simulink model "turbo_controller"  (R2025a)
settings: Solver=FixedStepAuto  StartTime=0.0  StopTime=inf  FixedStep=0.001  RelTol=1e-3
PostLoadFcn:
  | % 自动定位同目录CubeMX文件；不需要外部初始化脚本。
  | codertarget.data.setParameterValue('turbo_controller','STM32CubeMX.ProjectFile',fullfile(fileparts(get_param('turbo_controller','FileName')),'turbo_f407.ioc'));
InitFcn:
  | % 中文说明：按原控制器字段与类型创建三组接口总线；控制参数已内嵌。
  | tc_names=["EValve_Cycle" "EValve_Open" "Eblast_Cycle" "Eblast_Open" "Motor_Cycle" "Motor_Open" "EValve_Enable" "Eblast_Enable" "Motor_Enable" "SWO_Firework" "SWO_BleedAir" "EngineState" "Flag_ECUReset_Clear" "Flag_ECUReset_Save" "Flag_Reset_Enable" "Accelerator" "Nc_dem" "Nc"]; tc_types=["uint16" "uint16" "uint16" "uint16" "uint16" "uint16" "uint8" "uint8" "uint8" "uint8" "uint8" "uint8" "uint8" "uint8" "uint8" "single" "single" "single"];
  | for tc_k=1:numel(tc_names)
  |  tc_e(tc_k)=Simulink.BusElement; tc_e(tc_k).Name=char(tc_names(tc_k)); tc_e(tc_k).DataType=char(tc_types(tc_k));
  | end
  | EngineControl_Out=Simulink.Bus; EngineControl_Out.DataScope='Exported'; EngineControl_Out.Elements=tc_e;
  | clear tc_e tc_names tc_types tc_k
  | tc_names=["savedata1" "savedata2" "savedata3" "savedata4" "savedata5" "savedata6" "savedata7" "savedata8" "savedata9" "savedata10" "savedata11" "savedata12" "savedata13" "savedata14" "savedata15" "savedata16" "savedata17" "savedata18" "savedata19" "savedata20" "savedata21" "savedata22" "savedata23" "savedata24" "savedata25"]; tc_types=["single" "single" "single" "single" "single" "single" "single" "single" "single" "single" "single" "single" "single" "single" "single" "single" "single" "single" "single" "single" "single" "single" "single" "single" "single"];
  | for tc_k=1:numel(tc_names)
  |  tc_e(tc_k)=Simulink.BusElement; tc_e(tc_k).Name=char(tc_names(tc_k)); tc_e(tc_k).DataType=char(tc_types(tc_k));
  | end
  | SaveData_Out=Simulink.Bus; SaveData_Out.DataScope='Exported'; SaveData_Out.Elements=tc_e;
  | clear tc_e tc_names tc_types tc_k
  | tc_names=["senddata1" "senddata2" "senddata3" "senddata4" "senddata5" "senddata6" "senddata7" "senddata8" "senddata9" "senddata10" "senddata11" "senddata12" "senddata13" "senddata14" "senddata15" "senddata16" "senddata17" "senddata18" "senddata19" "senddata20" "senddata21" "senddata22" "senddata23" "senddata24" "senddata25" "senddata26" "senddata27" "senddata28" "senddata29"]; tc_types=["uint8" "uint8" "uint8" "uint8" "uint8" "uint8" "uint8" "uint8" "uint8" "uint8" "uint8" "uint8" "uint8" "uint8" "uint8" "uint8" "uint8" "uint8" "uint8" "uint8" "uint8" "uint8" "uint8" "uint8" "uint8" "uint8" "uint8" "uint8" "uint8"];
  | for tc_k=1:numel(tc_names)
  |  tc_e(tc_k)=Simulink.BusElement; tc_e(tc_k).Name=char(tc_names(tc_k)); tc_e(tc_k).DataType=char(tc_types(tc_k));
  | end
  | SendData_Out=Simulink.Bus; SendData_Out.DataScope='Exported'; SendData_Out.Elements=tc_e;
  | clear tc_e tc_names tc_types tc_k
  | 
  | % 以下为接口中文说明；只设置描述，不改变数值或数据类型。
  | EngineControl_Out.Description='执行控制输出（阀、电机、点火、状态及复位请求）';
  | tc_cn=["EValve_Cycle（主油阀周期计数（每计数2毫秒））" "EValve_Open（主油阀开通计数（每计数2毫秒））" "Eblast_Cycle（副油阀周期计数（每计数2毫秒））" "Eblast_Open（副油阀开通计数（每计数2毫秒））" "Motor_Cycle（起动电机周期计数）" "Motor_Open（起动电机开通计数）" "EValve_Enable（主油阀驱动使能）" "Eblast_Enable（副油阀驱动使能）" "Motor_Enable（起动电机使能）" "SWO_Firework（点火器使能（1开））" "SWO_BleedAir（引气阀使能（1开））" "EngineState（发动机状态）" "Flag_ECUReset_Clear（清除复位恢复状态请求）" "Flag_ECUReset_Save（保存复位恢复数据请求）" "Flag_Reset_Enable（处理器软件复位请求）" "Accelerator（油门／油泵给定控制量）" "Nc_dem（控制目标转速）" "Nc（发动机反馈转速（转每分））"];
  | tc_elements=EngineControl_Out.Elements;
  | for tc_k=1:numel(tc_cn)
  |  tc_elements(tc_k).Description=char(tc_cn(tc_k));
  | end
  | EngineControl_Out.Elements=tc_elements;
  | clear tc_cn tc_elements tc_k
  | SaveData_Out.Description='25项运行记录；字段含义按当前模型数据来源解释';
  | tc_cn=["savedata1（指令回显记录）" "savedata2（入口总温记录（℃））" "savedata3（电源电压记录）" "savedata4（排气温度记录（℃））" "savedata5（标定燃油压力记录）" "savedata6（副油阀占空比记录（％））" "savedata7（主油阀占空比记录（％））" "savedata8（温度修正转速记录）" "savedata9（开关输出及反馈位域）" "savedata10（物理转速记录）" "savedata11（油泵目标给定原始值）" "savedata12（起动电机占空比记录（％））" "savedata13（发动机状态码记录）" "savedata14（故障告警位域记录）" "savedata15（模型记录帧序号）" "savedata16（处理器温度记录（℃））" "savedata17（装订转速记录（沿用旧电源字段名））" "savedata18（导航高度记录）" "savedata19（飞行空速记录）" "savedata20（主阀旧记录位（恒零保留））" "savedata21（第21项保留记录（恒零））" "savedata22（保留记录项22）" "savedata23（保留记录项23）" "savedata24（保留记录项24）" "savedata25（保留记录项25）"];
  | tc_elements=SaveData_Out.Elements;
  | for tc_k=1:numel(tc_cn)
  |  tc_elements(tc_k).Description=char(tc_cn(tc_k));
  | end
  | SaveData_Out.Elements=tc_elements;
  | clear tc_cn tc_elements tc_k
  | SendData_Out.Description='29字段回传及外设命令接口；板端上位机帧只取第3至27字段';
  | tc_cn=["senddata1（回传发送允许标志（不直接上线路））" "senddata2（回传载荷长度25字节）" "senddata3（回传指令回显字节）" "senddata4（总温编码字节（℃＋80））" "senddata5（电源电压编码字节）" "senddata6（排温编码高字节）" "senddata7（排温编码低字节）" "senddata8（燃油压力编码高字节）" "senddata9（燃油压力编码低字节）" "senddata10（副油阀占空比字节（％））" "senddata11（主油阀占空比字节（％））" "senddata12（修正转速编码高字节）" "senddata13（修正转速编码低字节）" "senddata14（驱动及反馈状态位域）" "senddata15（物理转速编码高字节）" "senddata16（物理转速编码低字节）" "senddata17（油泵目标给定高字节（串口二使用））" "senddata18（油泵目标给定低字节（串口二使用））" "senddata19（起动电机占空比命令（串口一使用））" "senddata20（发动机状态码字节）" "senddata21（故障告警位域字节）" "senddata22（帧序号占位（板端另行填写））" "senddata23（处理器温度编码（℃＋50））" "senddata24（控制目标转速编码高字节）" "senddata25（控制目标转速编码低字节）" "senddata26（占位字节（板端改填实测泵速高字节））" "senddata27（占位字节（板端改填实测泵速低字节））" "senddata28（装订转速高字节（本板未发送））" "senddata29（装订转速低字节（本板未发送））"];
  | tc_elements=SendData_Out.Elements;
  | for tc_k=1:numel(tc_cn)
  |  tc_elements(tc_k).Description=char(tc_cn(tc_k));
  | end
  | SendData_Out.Elements=tc_elements;
  | clear tc_cn tc_elements tc_k
  | 
  | 
  | % FRAM模块化事务：接口类型和上电初始状态，随模型保存，无外部初始化文件。
  | clear FM_elements
  | FM_elements(1)=Simulink.BusElement;FM_elements(1).Name='phase';FM_elements(1).DataType='uint8';FM_elements(1).Dimensions=[1 1];FM_elements(1).Description='phase（当前事务阶段）';
  | FM_elements(2)=Simulink.BusElement;FM_elements(2).Name='a';FM_elements(2).DataType='uint8';FM_elements(2).Dimensions=[64 1];FM_elements(2).Description='a（启动时缓存的首区64字节）';
  | FM_elements(3)=Simulink.BusElement;FM_elements(3).Name='active';FM_elements(3).DataType='uint16';FM_elements(3).Dimensions=[1 1];FM_elements(3).Description='active（当前有效记录区地址）';
  | FM_elements(4)=Simulink.BusElement;FM_elements(4).Name='generation';FM_elements(4).DataType='uint32';FM_elements(4).Dimensions=[1 1];FM_elements(4).Description='generation（当前有效记录代号）';
  | FM_elements(5)=Simulink.BusElement;FM_elements(5).Name='record';FM_elements(5).DataType='uint8';FM_elements(5).Dimensions=[64 1];FM_elements(5).Description='record（本次冻结的待写记录）';
  | FM_elements(6)=Simulink.BusElement;FM_elements(6).Name='addr';FM_elements(6).DataType='uint16';FM_elements(6).Dimensions=[1 1];FM_elements(6).Description='addr（本次备用写入地址）';
  | FM_elements(7)=Simulink.BusElement;FM_elements(7).Name='lastSave';FM_elements(7).DataType='single';FM_elements(7).Dimensions=[1 1];FM_elements(7).Description='lastSave（上次开始保存的秒数）';
  | FM_elements(8)=Simulink.BusElement;FM_elements(8).Name='lastState';FM_elements(8).DataType='uint8';FM_elements(8).Dimensions=[1 1];FM_elements(8).Description='lastState（上次保存时的发动机状态）';
  | FM_elements(9)=Simulink.BusElement;FM_elements(9).Name='boot';FM_elements(9).DataType='boolean';FM_elements(9).Dimensions=[1 1];FM_elements(9).Description='boot（启动记录是否允许恢复）';
  | FM_elements(10)=Simulink.BusElement;FM_elements(10).Name='consumed';FM_elements(10).DataType='boolean';FM_elements(10).Dimensions=[1 1];FM_elements(10).Description='consumed（本次启动恢复通知是否已发送）';
  | FM_elements(11)=Simulink.BusElement;FM_elements(11).Name='payload';FM_elements(11).DataType='uint8';FM_elements(11).Dimensions=[20 1];FM_elements(11).Description='payload（当前20字节恢复内容）';
  | ... (+35 lines)
model workspace (MAT data in the model file):
  CRC16_Table_Reference = [0 4129 8258 12387 16516 20645 24774 28903 33032 37161 41290 45419 ... (256 elements, 256x1)]
  PE_Kaer = [0.15402 0.15402 0.12264 0.10076 0.09481 0.07601 0.07111 0.0569 0.05198 0.04926 0.05308 0.04325 ... (13 elements, 1x13)]
  PE_Nr = [21.2982 61.4260372 67.7475458 72.7394382 76.845934 80.6988798 83.8449282 86.6491912 88.9382406 89.178606 91.1938214 93.4068058 ... (13 elements, 1x13)]
  PE_Pump_Translate = 33.5999984741
  PE_RotaSpeed_Translate = 860
  PE_Taer = [0.4939154 0.4939154 0.40780982 0.34066978 0.31622756 0.30405716 0.34300244 0.26785022 0.37393554 0.23914836 0.44563948 0.31044662 ... (13 elements, 1x13)]
  PF_ACCFULLRANGE = 3360
  PF_Flag_ECUReset = 0
  PF_Flag_rx_suc = 1
  PF_Gear_Info = [40000; 45000; 50000; 55000; 57000; 59000; 60000; 61000; 61000; 61000; 61000; 61000]
  PF_K_TiaoJie = 1
  PF_Kpu = 10
  PF_MySet_Rxdata = [0 0 0 0 0 0 0 0 0 0 0 0 ... (50 elements, 50x1)]
  PF_MyUsart1_Rxdata = [0 0 0 0 0 0 0 0 0 0 0 0 ... (50 elements, 50x1)]
  PF_MyUsart2_Rxdata = [0 0 0 0 0 0 0 0 0 0 0 0 ... (50 elements, 50x1)]
  PF_Reset_Information = [0 0 0 0 0 0 0 0 0 0 0 0 ... (20 elements, 20x1)]
  PF_Sensor_X1_T4 = [0 4095]
  PF_Sensor_X2_T4 = [0 1.66666698456]
  PF_Sensor_X3_T4 = [0 504 999 1497 2010 2529 3051 3568 4076 4571 4959]
  PF_Sensor_X_P2 = [0.5 3]
  PF_Sensor_X_Poil = [0.5 3]
  PF_Sensor_X_T1t = [-50 300]
  PF_Sensor_X_Vpower = [0 3]
  PF_Sensor_X_Vpump = [0 3]
  PF_Sensor_Y1_T4 = [0 3]
  PF_Sensor_Y2_T4 = [0 5000]
  PF_Sensor_Y3_T4 = [0 100 200 300 400 500 600 700 800 900 980]
  PF_Sensor_Y_P2 = [0 1000]
  PF_Sensor_Y_Poil = [0 1000]
  PF_Sensor_Y_T1t = [-50 300]
  PF_Sensor_Y_Vpower = [0 33]
  PF_Sensor_Y_Vpump = [0 33]
  PG_CtrlMode_CloseLoop : mpt.Parameter (value not decoded)
  PG_CtrlMode_ManualAcc : mpt.Parameter (value not decoded)
  PG_CtrlMode_Origin : mpt.Parameter (value not decoded)
  PG_CtrlMode_Start : mpt.Parameter (value not decoded)
  PG_CtrlMode_Stop : mpt.Parameter (value not decoded)
  PG_ES_Clp : mpt.Parameter (value not decoded)
  PG_ES_EngStart : mpt.Parameter (value not decoded)
  PG_ES_Manual : mpt.Parameter (value not decoded)
  PG_ES_Origin : mpt.Parameter (value not decoded)
  PG_ES_Stop : mpt.Parameter (value not decoded)
  PG_Instr_BleedAirSet : mpt.Parameter (value not decoded)
  PG_Instr_CloseLoop : mpt.Parameter (value not decoded)
  PG_Instr_ECUReSet : mpt.Parameter (value not decoded)
  PG_Instr_EValveSet : mpt.Parameter (value not decoded)
  PG_Instr_EblastSet : mpt.Parameter (value not decoded)
  PG_Instr_Erase : mpt.Parameter (value not decoded)
  PG_Instr_FireWorkSet : mpt.Parameter (value not decoded)
  PG_Instr_ManualPlus : mpt.Parameter (value not decoded)
  PG_Instr_ManualrReduce : mpt.Parameter (value not decoded)
  PG_Instr_MotorSet : mpt.Parameter (value not decoded)
  PG_Instr_OilSet : mpt.Parameter (value not decoded)
  PG_Instr_SelfCheck : mpt.Parameter (value not decoded)
  PG_Instr_Start : mpt.Parameter (value not decoded)
  PG_Instr_Stop : mpt.Parameter (value not decoded)
  PG_Instr_StopZero : Simulink.Parameter (value not decoded)
  PG_Location_Air : Simulink.Parameter (value not decoded)
  PG_Location_Gnd : Simulink.Parameter (value not decoded)
  PG_ServoCtrlMode_CloseLoop : Simulink.Parameter (value not decoded)
  PG_ServoCtrlMode_CloseLoopMax : Simulink.Parameter (value not decoded)
  PG_ServoCtrlMode_CloseLoopMin : Simulink.Parameter (value not decoded)
  PG_ServoCtrlMode_ManualAcc : Simulink.Parameter (value not decoded)
  PG_ServoCtrlMode_ManualAccMax : Simulink.Parameter (value not decoded)
  PG_ServoCtrlMode_ManualAccMin : Simulink.Parameter (value not decoded)
  PG_SpeedDot_Permit : Simulink.Parameter (value not decoded)
  PL_EngineModel_Actuator = [0 10 100]
  PL_EngineModel_EngineStar_Press_P2 = [1013 1098.4 1099.144828 1099.931034 1103.613793 1162.662069 1143.793103 1131.006897 1123.186207 1117.6 1114 1111.806897 ... (127 elements, 1x127)]
  PL_EngineModel_EngineStar_RotaSpeed = [200 2000 9584 9660 10220 10240 10260 10288 10308 10368 10380 10408 ... (127 elements, 1x127)]
  PL_EngineModel_EngineStar_Temp_Exhaust = [128 129 129.1 130 131 131.1 132 133 134 134.1 135 135.1 ... (127 elements, 1x127)]
  PL_EngineModel_EngineStar_Time = [0.05 0.1 0.15 0.2 0.25 0.3 0.35 0.4 0.45 0.5 0.55 0.6 ... (127 elements, 1x127)]
  PL_EngineModel_IdleAbove_Nr = [0 21.2982 61.4260372 67.7475458 72.7394382 76.845934 80.6988798 83.8449282 86.6491912 88.9382406 89.178606 91.1938214 ... (14 elements, 1x14)]
  PL_EngineModel_IdleAbove_P2r = [0.986923266716 1.57907722675 1.81593881076 1.99358499877 2.23044658278 2.43770046879 2.65482358747 2.84233900814 3.03972366149 3.18776215149 3.25684678016 3.3950160375 ... (14 elements, 1x14)]
  PL_EngineModel_IdleAbove_Tempr = [0.0536001429337 1.07200285867 1.63301768805 1.63659103091 1.66875111667 1.72592460247 1.77595140254 1.86171163123 1.95461854565 2.03323208862 2.03323208862 2.13685903162 ... (14 elements, 1x14)]
  PL_EngineModel_IdleAbove_Ter = [0.42434128 0.42434128 0.42434128 0.30669408 0.23570008 0.22150128 0.1997974 0.23803274 0.16115638 0.24279948 0.13600422 0.31308354 ... (14 elements, 1x14)]
  PL_EngineModel_IdleAbove_Wfr = [0 10.142 23.8337 27.8905 31.9473 36.0041 40.0609 44.1177 48.1745 52.2313 52.7384 56.7952 ... (14 elements, 1x14)]
  PL_EngineModel_Press_P2 = [400 400 400 400 400 400 400 400 400 400]
  PL_EngineModel_Rotaspeed = [0 20000 96400]
  PL_EngineModel_Temp_Exhaust = [500 500 500 500 500 500 500 500 500 500]
  PL_Kaer = [0.1 0.1 0.1 0.1 0.1 0.1]
  PL_Nr = [50 60 70 80 90 100]
  PL_Taer = [0.1 0.1 0.1 0.1 0.1 0.1]
  Sig : Simulink.Signal (value not decoded)
  Ts_ms : Simulink.Parameter (value not decoded)
  false : Simulink.Parameter (value not decoded)
  true : Simulink.Parameter (value not decoded)
symbols that are objects in the model workspace (value not decoded): PG_CtrlMode_CloseLoop, PG_CtrlMode_ManualAcc, PG_CtrlMode_Origin, PG_CtrlMode_Start, PG_CtrlMode_Stop, PG_ES_Clp, PG_ES_EngStart, PG_ES_Manual, PG_ES_Origin, PG_ES_Stop, PG_Instr_BleedAirSet, PG_Instr_CloseLoop, PG_Instr_EblastSet, PG_Instr_ECUReSet, PG_Instr_Erase, PG_Instr_EValveSet, PG_Instr_FireWorkSet, PG_Instr_ManualPlus, PG_Instr_ManualrReduce, PG_Instr_MotorSet, PG_Instr_OilSet, PG_Instr_SelfCheck, PG_Instr_Start, PG_Instr_Stop, PG_Instr_StopZero, PG_ServoCtrlMode_CloseLoop, PG_ServoCtrlMode_CloseLoopMax, PG_ServoCtrlMode_CloseLoopMin, PG_ServoCtrlMode_ManualAcc, PG_ServoCtrlMode_ManualAccMax, PG_ServoCtrlMode_ManualAccMin, Ts_ms
libraries: simulink x97, stm32blockslib x10, stm32f4xxblockslib x8
(part 14 of 26)

== system turbo_controller/CLM/Manual/ManualAcc_Min_Control ==
  note: 形成手动油泵给定，并限制直接设定的范围
      |
      | 接收有效的手动直接设定命令时，把Data6限制在0～70，再乘以100，形成泵控制编码。例：Data6=35
      | 得到3500，Data6=90会先限制为70，输出7000。这是设备控制编码，不是油压或燃油流量。
      |
      | 没有直接设定命令时，使用“手动加减”分支产生的保持值。选择器决定采用新设定还是保持路径，范
      | 围模块防止结果超出允许值。对外同时给出手动控制上下界0和15000，供后续统一输出处理。最终泵命
      | 令还会经过使能、限幅和字节打包，才发送到泵。
  S_Flag_rs_suc : Inport
      settings: AttributesFormatString=S_Flag_rs_suc（标志接收状态成功或有效）
  S_Instr : Inport  Port=2
      settings: AttributesFormatString=S_Instr（指令）
  S_ServoOut_Last : Inport  Port=3
      settings: AttributesFormatString=S_ServoOut_Last（伺服输出上一周期）
  S_COMM_Data6 : Inport  Port=4
      settings: AttributesFormatString=S_COMM_Data6（通信数据6）
  S_OverSpeed_Protect : Inport  Port=5
      settings: AttributesFormatString=S_OverSpeed_Protect（超速保护）
  Bus Selector2 : BusSelector  OutputSignals=Accelerator（油泵给定控制量）
      settings: AttributesFormatString=Bus Selector2（总线选择器2）
  Constant1 : Constant  Value=0  OutDataTypeStr=single
      settings: AttributesFormatString=Constant1（常量1）
  Constant2 : Constant  Value=100  OutDataTypeStr=single
      settings: AttributesFormatString=Constant2（常量2）
  Constant3 : Constant  Value=70  OutDataTypeStr=single
      settings: AttributesFormatString=Constant3（常量3）
  Constant4 : Constant  Value=0  OutDataTypeStr=single
      settings: AttributesFormatString=Constant4（常量4）
  Constant5 : Constant  Value=10000  OutDataTypeStr=single
      settings: AttributesFormatString=Constant5（常量5）
  Constant6 : Constant  Value=15000  OutDataTypeStr=single
      settings: AttributesFormatString=Constant6（常量6）
  Data Type Conversion2 : DataTypeConversion  OutDataTypeStr=single  SaturateOnIntegerOverflow=off  RndMeth=Floor
      settings: AttributesFormatString=Data Type Conversion2（数据类型转换2）
  LogicSelection1 : Subsystem  Description=|  RTWFcnName=LogicSelF  RTWFileName=EngineControl_GeneralModule
      | 在“采用新设定”和“保持旧设定”之间选择
      | 
      | C是选择条件，T是条件成立时要采用的新值，F是条件不成立时保留的值。C不为0输出T，C为0输出F。这里不是三个数参与计算，也不把T、F相加。
      | 
      | 在手动油泵父系统里，它用于决定是否接受本次命令。例如新设定3500、原设定3200：条件有效输出3500，条件无效仍输出3200。本模块自身没有存储，旧值由外部反馈提供。
      settings: AttributesFormatString=LogicSelection1（逻辑选择1）  RTWFcnNameOpts=User specified  RTWFileNameOpts=User specified
  Logical Operator : Logic  AllPortsSameDT=off  OutDataTypeStr=boolean
      settings: AttributesFormatString=Logical Operator（逻辑运算）
  N1r_idle1 : Constant  Value=PG_Instr_OilSet  OutDataTypeStr=single  SampleTime=-1
      settings: AttributesFormatString=N1r_idle1（一级转速归一化值慢车1）
  Product2 : Product  Inputs=**/
      settings: AttributesFormatString=Product2（乘法2）
  Range : Stateflow chart  Description=|  TreatAsAtomicUnit=on
      | 本实例把手动Data6限制在0～70，随后父级乘100变成泵给定0～7000。例如输入90先变70，再得到7000。
      | 
      | 把一个数限制在允许范围内
      | 
      | 输入包括待处理值、允许下限和允许上限。先比较是否越过上限，越过就输出上限；未超过上限时再检查下限，小于下限就输出下限；落在范围内则原样通过。恰好等于边界的值也保留。
      | 
      | 计算式：输出 = min(max(输入，下限)，上限)。
      | 例如下限为0、上限为100时，输入120输出100，输入-5输出0，输入60输出60。这里不做平均、不计算变化速度，也不记住上一拍；它只防止当前数值越界。具体边界由父子系统连入，不能把此处的输出一律理解为百分比。
      settings: AttributesFormatString=Range（限幅或范围）
  Relational Operator1 : RelationalOperator  Operator===  OutDataTypeStr=boolean  InputSameDT=off
      settings: AttributesFormatString=Relational Operator1（关系比较运算1）
  手动加减 : Subsystem  Description=|
      | 处理手动加、减命令，并让按键作用保持一段时间
      | 
      | 本分支读取命令和上次油泵给定。有效的加命令产生“旧值+100”，减命令产生“旧值-100”；其余命令保持旧值。超速保护成立时，优先走减100路径。
      | 
      | Hold_500ms把触发后的操作状态维持指定时间，父级据此选择更新或保持。它的内部时间换算使用Time_ms/Ts_ms；当前Ts_ms=20 ms，因此500 ms对应25次调用。名称中的500 ms表示保持窗口，不意味着每个20 ms都能无限叠加一次命令。最终值仍受父级限幅约束。
  S_ManualAcc : Outport
      settings: AttributesFormatString=S_ManualAcc（手动油门）
  S_ManualAcc_Min : Outport  Port=2
      settings: AttributesFormatString=S_ManualAcc_Min（手动油门下限）
  S_ManualAcc_Max : Outport  Port=3
      settings: AttributesFormatString=S_ManualAcc_Max（手动油门上限）
  wires:
  Constant5/1 -> Product2/1
  S_COMM_Data6/1 -> Data Type Conversion2/1
  S_Instr/1 -> 手动加减/2(In2), Relational Operator1/2
  S_ServoOut_Last/1 -> Bus Selector2/1
  手动加减/1(Out2) -> LogicSelection1/2(F)
  S_Flag_rs_suc/1 -> 手动加减/1(In1), Logical Operator/2
  Logical Operator/1 -> LogicSelection1/1(C)
  N1r_idle1/1 -> Relational Operator1/1
  Relational Operator1/1 -> Logical Operator/1
  Product2/1 -> LogicSelection1/3(T)
  Constant2/1 -> Product2/3
  LogicSelection1/1(Out) -> S_ManualAcc/1
  Constant1/1 -> Range/3(Min)
  Constant3/1 -> Range/2(Max)
  Range/1(Out) -> Product2/2
  Data Type Conversion2/1 -> Range/1(In)
  Constant4/1 -> S_ManualAcc_Min/1
  Constant6/1 -> S_ManualAcc_Max/1
  Bus Selector2/1 -> 手动加减/3(In3)  "<Accelerator（油泵给定控制量）>"
  S_OverSpeed_Protect/1 -> 手动加减/4(In4)

== system turbo_controller/CLM/Manual/ManualEValve_Control ==
  note: 把手动油阀开度换算为周期内的开通拍数
      |
      | 先确认有效帧属于本阀的设置命令，再把命令数据Data6按百分数换算：开通计数 = Data6×30/100，并
      | 限制在0～30；周期固定为30。例：Data6=50得到开通15拍，Data6=100得到开通30拍。
      |
      | 使能判断使用换算后的计数是否大于等于1，因此非常小的设定可能仍不使能阀门。没有本阀的新有效
      | 设置时，保持原设定。本处只生成周期、开通和使能三项，实际的2 ms输出节拍在板级输出中执行。
      |
      | 若阀门周期30、开通15，在2 ms节拍下就是每60 ms开30 ms。不要把这里的“15”直接读成15 ms。
  S_Flag_rs_suc : Inport
      settings: AttributesFormatString=S_Flag_rs_suc（标志接收状态成功或有效）
  S_Instr : Inport  Port=2
      settings: AttributesFormatString=S_Instr（指令）
  S_COMM_Data6 : Inport  Port=3
      settings: AttributesFormatString=S_COMM_Data6（通信数据6）
  S_ServoOut_Last : Inport  Port=4
      settings: AttributesFormatString=S_ServoOut_Last（伺服输出上一周期）
  Bus Selector2 : BusSelector  OutputSignals=EValve_Open（主油阀开通计数）,EValve_Enable（主油阀使能）
      settings: AttributesFormatString=Bus Selector2（总线选择器2）
  Constant1 : Constant  Value=0  OutDataTypeStr=single
      settings: AttributesFormatString=Constant1（常量1）
  Constant2 : Constant  Value=100  OutDataTypeStr=single
      settings: AttributesFormatString=Constant2（常量2）
  Constant3 : Constant  Value=30  OutDataTypeStr=single
      settings: AttributesFormatString=Constant3（常量3）
  Constant5 : Constant  Value=30  OutDataTypeStr=uint16
      settings: AttributesFormatString=Constant5（常量5）
  Constant7 : Constant  Value=30  OutDataTypeStr=single
      settings: AttributesFormatString=Constant7（常量7）
  Constant8 : Constant  OutDataTypeStr=single
      settings: AttributesFormatString=Constant8（常量8）
  Data Type Conversion1 : DataTypeConversion  OutDataTypeStr=uint16  SaturateOnIntegerOverflow=off  RndMeth=Floor
      settings: AttributesFormatString=Data Type Conversion1（数据类型转换1）
  Data Type Conversion2 : DataTypeConversion  OutDataTypeStr=single  SaturateOnIntegerOverflow=off  RndMeth=Floor
      settings: AttributesFormatString=Data Type Conversion2（数据类型转换2）
  Data Type Conversion3 : DataTypeConversion  OutDataTypeStr=uint8  SaturateOnIntegerOverflow=off  RndMeth=Floor
      settings: AttributesFormatString=Data Type Conversion3（数据类型转换3）
  Logical Operator : Logic  AllPortsSameDT=off  OutDataTypeStr=boolean
      settings: AttributesFormatString=Logical Operator（逻辑运算）
  N1r_idle1 : Constant  Value=PG_Instr_EValveSet  OutDataTypeStr=single  SampleTime=-1
      settings: AttributesFormatString=N1r_idle1（一级转速归一化值慢车1）
  Product3 : Product  Inputs=*/*
      settings: AttributesFormatString=Product3（乘法3）
  Range : Stateflow chart  Description=|  TreatAsAtomicUnit=on
      | 本实例限制主油阀开通计数0～30。周期固定30，换算值15表示半周期开通；板级2 ms节拍下对应开30 ms、关30 ms。
      | 
      | 把一个数限制在允许范围内
      | 
      | 输入包括待处理值、允许下限和允许上限。先比较是否越过上限，越过就输出上限；未超过上限时再检查下限，小于下限就输出下限；落在范围内则原样通过。恰好等于边界的值也保留。
      | 
      | 计算式：输出 = min(max(输入，下限)，上限)。
      | 例如下限为0、上限为100时，输入120输出100，输入-5输出0，输入60输出60。这里不做平均、不计算变化速度，也不记住上一拍；它只防止当前数值越界。具体边界由父子系统连入，不能把此处的输出一律理解为百分比。
      settings: AttributesFormatString=Range（限幅或范围）
  Relational Operator1 : RelationalOperator  Operator===  OutDataTypeStr=boolean  InputSameDT=off
      settings: AttributesFormatString=Relational Operator1（关系比较运算1）
  Relational Operator2 : RelationalOperator  OutDataTypeStr=boolean  InputSameDT=off
      settings: AttributesFormatString=Relational Operator2（关系比较运算2）
  Switch : Switch  Criteria=u2 ~= 0  SaturateOnIntegerOverflow=off  InputSameDT=off
      settings: AttributesFormatString=Switch（开关选择）
  Switch1 : Switch  Criteria=u2 ~= 0  SaturateOnIntegerOverflow=off  InputSameDT=off
      settings: AttributesFormatString=Switch（开关选择）
  S_EValve_Cycle : Outport
      settings: AttributesFormatString=S_EValve_Cycle（主油阀周期计数（每计数2毫秒））
  S_EValve_Open : Outport  Port=2
      settings: AttributesFormatString=S_EValve_Open（主油阀开通计数（每计数2毫秒））
  S_EValve_Enable : Outport  Port=3
      settings: AttributesFormatString=S_EValve_Enable（主油阀驱动使能）
  wires:
  S_COMM_Data6/1 -> Data Type Conversion2/1
  S_Instr/1 -> Relational Operator1/2
  S_Flag_rs_suc/1 -> Logical Operator/2
  N1r_idle1/1 -> Relational Operator1/1
  Relational Operator1/1 -> Logical Operator/1
  Switch/1 -> S_EValve_Open/1
  Constant1/1 -> Range/3(Min)
  Constant3/1 -> Range/2(Max)
  Data Type Conversion2/1 -> Product3/1
  Constant5/1 -> S_EValve_Cycle/1
  Range/1(Out) -> Data Type Conversion1/1
  Constant2/1 -> Product3/2
  Product3/1 -> Range/1(In), Relational Operator2/1
  Constant7/1 -> Product3/3
  Bus Selector2/1 -> Switch/3  "<EValve_Open（主油阀开通计数）>"
  Switch1/1 -> Data Type Conversion3/1
  Constant8/1 -> Relational Operator2/2
  Bus Selector2/2 -> Switch1/3  "<EValve_Enable（主油阀使能）>"
  Data Type Conversion3/1 -> S_EValve_Enable/1
  S_ServoOut_Last/1 -> Bus Selector2/1
  Data Type Conversion1/1 -> Switch/1
  Relational Operator2/1 -> Switch1/1
  Logical Operator/1 -> Switch1/2, Switch/2

== system turbo_controller/CLM/Manual/Motor_Control ==
  note: 把手动命令转换为起动电机开通设定
      |
      | 只有有效帧且命令属于电机设置时才更新。Data6直接作为开通计数，限制为0～100；周期固定100。原
      | 数据达到1才设置电机使能，否则关闭。
      |
      | 例如Data6=40表示100个节拍中开40拍，不表示40 rpm。未收到相应命令时使用延迟记住上次的周期、
      | 开通和使能。结果由输出管理与板级时序继续处理，本模块不读取电机实际转速，也不进行速度闭环。
  S_Flag_rs_suc : Inport
      settings: AttributesFormatString=S_Flag_rs_suc（标志接收状态成功或有效）
  S_Instr : Inport  Port=2
      settings: AttributesFormatString=S_Instr（指令）
  S_COMM_Data6 : Inport  Port=3
      settings: AttributesFormatString=S_COMM_Data6（通信数据6）
  Constant1 : Constant  Value=0  OutDataTypeStr=single
      settings: AttributesFormatString=Constant1（常量1）
  Constant3 : Constant  Value=100  OutDataTypeStr=single
      settings: AttributesFormatString=Constant3（常量3）
  Constant5 : Constant  Value=100  OutDataTypeStr=uint16
      settings: AttributesFormatString=Constant5（常量5）
  Constant8 : Constant  OutDataTypeStr=single
      settings: AttributesFormatString=Constant8（常量8）
  Data Type Conversion1 : DataTypeConversion  OutDataTypeStr=uint16  SaturateOnIntegerOverflow=off  RndMeth=Floor
      settings: AttributesFormatString=Data Type Conversion1（数据类型转换1）
  Data Type Conversion2 : DataTypeConversion  OutDataTypeStr=single  SaturateOnIntegerOverflow=off  RndMeth=Floor
      settings: AttributesFormatString=Data Type Conversion2（数据类型转换2）
  Data Type Conversion3 : DataTypeConversion  OutDataTypeStr=uint8  SaturateOnIntegerOverflow=off  RndMeth=Floor
      settings: AttributesFormatString=Data Type Conversion3（数据类型转换3）
  Logical Operator : Logic  AllPortsSameDT=off  OutDataTypeStr=boolean
      settings: AttributesFormatString=Logical Operator（逻辑运算）
  N1r_idle1 : Constant  Value=PG_Instr_MotorSet  OutDataTypeStr=single  SampleTime=-1
      settings: AttributesFormatString=N1r_idle1（一级转速归一化值慢车1）
  Range : Stateflow chart  Description=|  TreatAsAtomicUnit=on
      | 本实例限制手动电机开通计数0～100，周期100。设定120只输出100，不会超过满周期；使能还由父级单独判断。
      | 
      | 把一个数限制在允许范围内
      | 
      | 输入包括待处理值、允许下限和允许上限。先比较是否越过上限，越过就输出上限；未超过上限时再检查下限，小于下限就输出下限；落在范围内则原样通过。恰好等于边界的值也保留。
      | 
      | 计算式：输出 = min(max(输入，下限)，上限)。
      | 例如下限为0、上限为100时，输入120输出100，输入-5输出0，输入60输出60。这里不做平均、不计算变化速度，也不记住上一拍；它只防止当前数值越界。具体边界由父子系统连入，不能把此处的输出一律理解为百分比。
      settings: AttributesFormatString=Range（限幅或范围）
  Relational Operator1 : RelationalOperator  Operator===  OutDataTypeStr=boolean  InputSameDT=off
      settings: AttributesFormatString=Relational Operator1（关系比较运算1）
  Relational Operator2 : RelationalOperator  OutDataTypeStr=boolean  InputSameDT=off
      settings: AttributesFormatString=Relational Operator2（关系比较运算2）
  Switch : Switch  Criteria=u2 ~= 0  SaturateOnIntegerOverflow=off  InputSameDT=off
      settings: AttributesFormatString=Switch（开关选择）
  Switch1 : Switch  Criteria=u2 ~= 0  SaturateOnIntegerOverflow=off  InputSameDT=off
      settings: AttributesFormatString=Switch（开关选择）
  Time Delay1 : UnitDelay  SampleTime=-1  HasFrameUpgradeWarning=on
      settings: AttributesFormatString=Time Delay1（时间延迟1）
  Time Delay8 : UnitDelay  SampleTime=-1  HasFrameUpgradeWarning=on
      settings: AttributesFormatString=Time Delay8（时间延迟8）
  S_Motor_Cycle : Outport
      settings: AttributesFormatString=S_Motor_Cycle（起动电机周期计数）
  S_Motor_Open : Outport  Port=2
      settings: AttributesFormatString=S_Motor_Open（起动电机开通计数）
  S_Motor_Enable : Outport  Port=3
      settings: AttributesFormatString=S_Motor_Enable（起动电机使能）
  wires:
  S_COMM_Data6/1 -> Data Type Conversion2/1
  S_Instr/1 -> Relational Operator1/2
  S_Flag_rs_suc/1 -> Logical Operator/2
  N1r_idle1/1 -> Relational Operator1/1
  Relational Operator1/1 -> Logical Operator/1
  Switch/1 -> Time Delay8/1, S_Motor_Open/1
  Constant1/1 -> Range/3(Min)
  Constant3/1 -> Range/2(Max)
  Constant5/1 -> S_Motor_Cycle/1
  Range/1(Out) -> Data Type Conversion1/1
  Data Type Conversion2/1 -> Range/1(In), Relational Operator2/1
  Switch1/1 -> Time Delay1/1, Data Type Conversion3/1
  Constant8/1 -> Relational Operator2/2
  Data Type Conversion3/1 -> S_Motor_Enable/1
  Time Delay8/1 -> Switch/3
  Data Type Conversion1/1 -> Switch/1
  Time Delay1/1 -> Switch1/3
  Relational Operator2/1 -> Switch1/1
  Logical Operator/1 -> Switch1/2, Switch/2

== system turbo_controller/CLM/Start/HoldFirst ==
  note: 保存进入起动时的排温和油压参考
      |
      | 起动前的T4、油压会在进入本分支时被锁住。Hold图提供首次运行标志，外面的开关和延迟负责保存对
      | 应的传感器数值；不是Hold图自己保存两路模拟量。
      |
      | 起动期间，即便当前排温或油压改变，参考值也保持进入时的水平。后面的起动图用“当前油压-起动
      | 前油压”判断压力是否建立。排温参考输出当前接Unused_OriginT4终止端，并未送入起动图；图内T4_
      | 01则在到达1000 rpm阶段另取当时排温。不能因为这里保持了两路，就认为两路都被采用。
  S_Origin_T4 : Inport
      settings: AttributesFormatString=S_Origin_T4（起动前保存的排温初值）
  S_Origin_POil : Inport  Port=2
      settings: AttributesFormatString=S_Origin_POil（起动前保存的燃油压力初值）
  Delay : Delay  DelayLength=1
      settings: AttributesFormatString=Delay（延迟）
  Delay1 : Delay  DelayLength=1
      settings: AttributesFormatString=Delay1（延迟1）
  Hold : Stateflow chart  Description=|  TreatAsAtomicUnit=on  RTWFcnName=Timmer  RTWFileName=EngineControl_Timmer
      | 识别本次执行的第一次调用
      | 
      | 内部保持一个首次标志。第一次进入时给出用于初始化的标志，之后把内部状态切换为已经执行，使后续调用采用保持或正常处理路径。
      | 
      | 本图自身不存储温度、油压或参数数组。需要保留的具体数值在父系统的开关与延迟中保存；本图只告诉父系统何时取初值。它也不是每拍都产生一次上升沿。重新初始化模型时会重新开始这一首次判断。
      settings: AttributesFormatString=Hold（保持）  RTWSystemCode=Reusable function  RTWFcnNameOpts=Use subsystem name  RTWFileNameOpts=User specified
  Switch : Switch  Criteria=u2 ~= 0  SaturateOnIntegerOverflow=off  InputSameDT=off
      settings: AttributesFormatString=Switch（开关选择）
  Switch1 : Switch  Criteria=u2 ~= 0  SaturateOnIntegerOverflow=off  InputSameDT=off
      settings: AttributesFormatString=Switch（开关选择）
  S_Origin_T4_0 : Outport
      settings: AttributesFormatString=S_Origin_T4_0（起动前保存的排温初值）
  S_Origin_POil_1 : Outport  Port=2
      settings: AttributesFormatString=S_Origin_POil_1（起动前保存的燃油压力初值）
  wires:
  Switch/1 -> Delay/1, S_Origin_T4_0/1
  Switch1/1 -> S_Origin_POil_1/1, Delay1/1
  Delay/1 -> Switch/3
  S_Origin_T4/1 -> Switch/1
  Hold/1(Out) -> Switch/2, Switch1/2
  S_Origin_POil/1 -> Switch1/1
  Delay1/1 -> Switch1/3

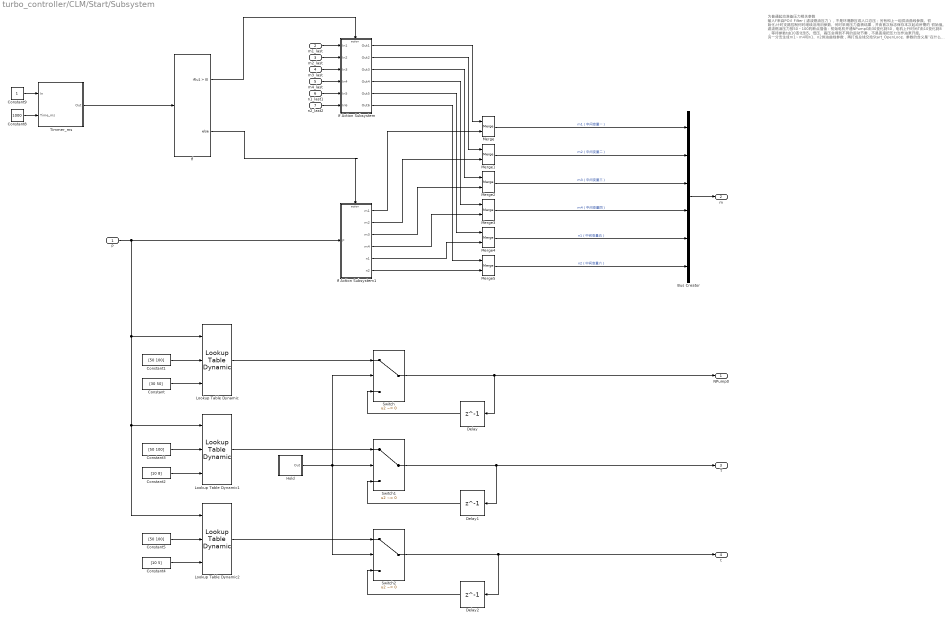
== system turbo_controller/CLM/Start/Subsystem ==
  note: 为普通起动准备压力相关参数
      |
      | 输入P来自POil_Filter（滤波燃油压力），不是环境静压或入口总压；另有和上一组供油曲线参数。初
      | 始化/计时支路控制何时继续沿用旧参数、何时采用压力查表结果，并由首次标志保存本次起动所需的
      | 初始值。
      |
      | 滤波燃油压力按50～100的断点插值：初始电机开通NPump0由30变化到50，电机上升时间T由10变化到8
      | ，等待参数t由10变化到5。低压、高压会得到不同的起动节奏，不是直接把压力当作油泵开度。
      |
      | 另一分支生成m1～m4和n1、n2供油曲线参数，再打成总线交给Start_OpenLoop。参数的含义是“在什么
      | 转速给多少泵编码、等待多久”，不代表实际油压已达到目标。
  P : Inport
      settings: AttributesFormatString=P（压力或比例变量）
  m1_last : Inport  Port=2
      settings: AttributesFormatString=m1_last（中位或中间变量1上一周期）
  m2_last : Inport  Port=3
      settings: AttributesFormatString=m2_last（中位或中间变量2上一周期）
  m3_last : Inport  Port=4
      settings: AttributesFormatString=m3_last（中位或中间变量3上一周期）
  m4_last : Inport  Port=5
      settings: AttributesFormatString=m4_last（中位或中间变量4上一周期）
  n1_last1 : Inport  Port=6
      settings: AttributesFormatString=n1_last1（转速变量1上一周期1）
  n2_last2 : Inport  Port=7
      settings: AttributesFormatString=n2_last2（转速变量2上一周期2）
  Bus Creator : BusCreator  Inputs=6
      settings: AttributesFormatString=Bus Creator（总线创建器）
  Constant : Constant  Value=[30 50]  OutDataTypeStr=uint16
      settings: AttributesFormatString=Constant（常量）
  Constant1 : Constant  Value=[50 100]  OutDataTypeStr=single
      settings: AttributesFormatString=Constant1（常量1）
  Constant2 : Constant  Value=[10 8]  OutDataTypeStr=uint16
      settings: AttributesFormatString=Constant2（常量2）
  Constant3 : Constant  Value=[50 100]  OutDataTypeStr=single
      settings: AttributesFormatString=Constant3（常量3）
  Constant4 : Constant  Value=[10 5]  OutDataTypeStr=uint16
      settings: AttributesFormatString=Constant4（常量4）
  Constant5 : Constant  Value=[50 100]  OutDataTypeStr=single
      settings: AttributesFormatString=Constant5（常量5）
  Constant8 : Constant  Value=1000  OutDataTypeStr=single
      settings: AttributesFormatString=Constant8（常量8）
  Constant9 : Constant  OutDataTypeStr=boolean
      settings: AttributesFormatString=Constant9（常量9）
  Delay : Delay  DelayLength=1
      settings: AttributesFormatString=Delay（延迟）
  Delay1 : Delay  DelayLength=1
      settings: AttributesFormatString=Delay1（延迟1）
  Delay2 : Delay  DelayLength=1
      settings: AttributesFormatString=Delay2（延迟2）
  Hold : Stateflow chart  Description=|  TreatAsAtomicUnit=on  RTWFcnName=Timmer  RTWFileName=EngineControl_Timmer
      | 识别本次执行的第一次调用
      | 
      | 内部保持一个首次标志。第一次进入时给出用于初始化的标志，之后把内部状态切换为已经执行，使后续调用采用保持或正常处理路径。
      | 
      | 本图自身不存储温度、油压或参数数组。需要保留的具体数值在父系统的开关与延迟中保存；本图只告诉父系统何时取初值。它也不是每拍都产生一次上升沿。重新初始化模型时会重新开始这一首次判断。
      settings: AttributesFormatString=Hold（保持）  RTWSystemCode=Reusable function  RTWFcnNameOpts=Use subsystem name  RTWFileNameOpts=User specified
  If : If
      settings: AttributesFormatString=If（如果）
  If Action Subsystem : Subsystem  Description=|  TreatAsAtomicUnit=on
      | 在参数切换前继续使用上一组起动曲线
      | 
      | 本分支把输入的m1、m2、m3、m4、n1、n2按原顺序打成参数总线，不改变其数值。上层条件选择本分支时，普通起动继续沿用此前保存的曲线。
      | 
      | 例如旧m1为1600，本分支仍输出1600，不会根据当前压力重新计算。压力查表更新在另一个动作分支完成；两条分支由父级If选择后汇合，不能把两组参数相加。
      settings: AttributesFormatString=If Action Subsystem（条件动作子系统）
  If Action Subsystem1 : Subsystem  Description=|  TreatAsAtomicUnit=on
      | 根据滤波燃油压力生成普通起动的供油曲线
      | 
      | 使用滤波燃油压力50和100两个断点线性插值。对应参数分别为：
      | m1：1600→1900；m2：1700→2500；
      | m3：1900→2700；m4：1500→2300；
      | n1：8800→7000；n2固定20000 rpm。
      | 
      | 例如压力处于两个断点正中间75时，m1=1750、m2=2100、m3=2300、m4=1900、n1=7900。m是泵控制编码，n是阶段转速参数。生成的六项打成一组送起动顺序图，后者再结合当前转速计算实际给定。
      settings: AttributesFormatString=If Action Subsystem1（条件动作子系统1）
  Lookup Table Dynamic : simulink/Lookup Tables/Lookup Table Dynamic  LookUpMeth=Interpolation-Use End Values  OutDataType=fixdt('uint16')  OutScaling=[]  OutputDataTypeScalingMode=Specify via dialog  OutDataTypeStr=fixdt('uint16')  DoSatur=off
      settings: AttributesFormatString=Lookup Table Dynamic（动态查表）
  Lookup Table Dynamic1 : simulink/Lookup Tables/Lookup Table Dynamic  LookUpMeth=Interpolation-Use End Values  OutDataType=fixdt('uint16')  OutScaling=[]  OutputDataTypeScalingMode=Specify via dialog  OutDataTypeStr=fixdt('uint16')  DoSatur=off
      settings: AttributesFormatString=Lookup Table Dynamic1（动态查表1）
  Lookup Table Dynamic2 : simulink/Lookup Tables/Lookup Table Dynamic  LookUpMeth=Interpolation-Use End Values  OutDataType=fixdt('uint16')  OutScaling=[]  OutputDataTypeScalingMode=Specify via dialog  OutDataTypeStr=fixdt('uint16')  DoSatur=off
      settings: AttributesFormatString=Lookup Table Dynamic2（动态查表2）
  Merge{,1..5} (6 alike) : Merge
      Merge settings: AttributesFormatString=Merge（条件分支输出合并）
      Merge1 settings: AttributesFormatString=Merge1（条件分支输出合并1）
      Merge2 settings: AttributesFormatString=Merge2（条件分支输出合并2）
      Merge3 settings: AttributesFormatString=Merge3（条件分支输出合并3）
      Merge4 settings: AttributesFormatString=Merge4（条件分支输出合并4）
      Merge5 settings: AttributesFormatString=Merge5（条件分支输出合并5）
  Switch : Switch  Criteria=u2 ~= 0  SaturateOnIntegerOverflow=off  InputSameDT=off
      settings: AttributesFormatString=Switch（开关选择）
  Switch1 : Switch  Criteria=u2 ~= 0  SaturateOnIntegerOverflow=off  InputSameDT=off
      settings: AttributesFormatString=Switch（开关选择）
  Switch2 : Switch  Criteria=u2 ~= 0  SaturateOnIntegerOverflow=off  InputSameDT=off
      settings: AttributesFormatString=Switch（开关选择）
  Timmer_ms : Stateflow chart  Description=|  TreatAsAtomicUnit=on  RTWFcnName=Timmer  RTWFileName=EngineControl_Timmer
      | 起动参数切换所用的毫秒定时器
      | 
      | 每次调用按Ts_ms所代表的时间推进计数，到Time_ms对应的调用次数时输出到时状态。当前控制节拍20 ms，1000 ms要累计50次调用，不能把内部计数50理解为50 s。
      | 
      | 父系统利用此状态决定继续沿用历史参数，还是切换到本次压力计算的参数。这里不读取压力，也不决定m1、m2等曲线值；它只提供参数切换的时间条件。
      settings: AttributesFormatString=Timmer_ms（计时器毫秒）  RTWSystemCode=Reusable function  RTWFcnNameOpts=Use subsystem name  RTWFileNameOpts=User specified
  NPump0 : Outport
      settings: AttributesFormatString=NPump0（油泵转速0）
  m : Outport  Port=2
      settings: AttributesFormatString=m（中间变量或中位）
  T : Outport  Port=3
      settings: AttributesFormatString=T（温度、时间或真分支输入）
  t : Outport  Port=4
      settings: AttributesFormatString=t（温度、时间或真分支输入）
  wires:
  Constant8/1 -> Timmer_ms/2(Time_ms)
  Constant9/1 -> Timmer_ms/1(In)
  Timmer_ms/1(Out) -> If/1
  If/1 -> If Action Subsystem/Action
  If/2 -> If Action Subsystem1/Action
  m1_last/1 -> If Action Subsystem/1(In1)
  If Action Subsystem/1(Out1) -> Merge/1
  If Action Subsystem1/1(m1) -> Merge/2
  m2_last/1 -> If Action Subsystem/2(In2)
  m3_last/1 -> If Action Subsystem/3(In3)
  m4_last/1 -> If Action Subsystem/4(In4)
  If Action Subsystem1/2(m2) -> Merge1/2
  If Action Subsystem1/3(m3) -> Merge2/2
  If Action Subsystem1/4(m4) -> Merge3/2
  If Action Subsystem/2(Out2) -> Merge1/1
  If Action Subsystem/3(Out3) -> Merge2/1
  If Action Subsystem/4(Out4) -> Merge3/1
  Bus Creator/1 -> m/1
  Merge/1 -> Bus Creator/1  "m1（中间变量一）"
  Merge1/1 -> Bus Creator/2  "m2（中间变量二）"
  Merge2/1 -> Bus Creator/3  "m3（中间变量三）"
  Merge3/1 -> Bus Creator/4  "m4（中间变量四）"
  Switch/1 -> NPump0/1, Delay/1
  Constant/1 -> Lookup Table Dynamic/3
  Constant1/1 -> Lookup Table Dynamic/2
  n1_last1/1 -> If Action Subsystem/5(In5)
  n2_last2/1 -> If Action Subsystem/6(In6)
  If Action Subsystem/5(Out5) -> Merge4/1
  If Action Subsystem1/5(n1) -> Merge4/2
  If Action Subsystem/6(Out6) -> Merge5/1
  If Action Subsystem1/6(n2) -> Merge5/2
  Merge4/1 -> Bus Creator/5  "n1（中间变量五）"
  Merge5/1 -> Bus Creator/6  "n2（中间变量六）"
  Switch1/1 -> T/1, Delay1/1
  Constant2/1 -> Lookup Table Dynamic1/3
  Constant3/1 -> Lookup Table Dynamic1/2
  P/1 -> Lookup Table Dynamic2/1, Lookup Table Dynamic1/1, Lookup Table Dynamic/1, If Action Subsystem1/1(P)
  Switch2/1 -> t/1, Delay2/1
  Constant4/1 -> Lookup Table Dynamic2/3
  Constant5/1 -> Lookup Table Dynamic2/2
  Delay1/1 -> Switch1/3
  Lookup Table Dynamic1/1 -> Switch1/1
  Delay2/1 -> Switch2/3
  Lookup Table Dynamic2/1 -> Switch2/1
  Hold/1(Out) -> Switch/2, Switch2/2, Switch1/2
  Delay/1 -> Switch/3
  Lookup Table Dynamic/1 -> Switch/1
